simulink model "rc_receiver"  (R2026b)
settings: Solver=VariableStepAuto
undefined symbols (not defined in the file or in its folder): DiscIntNeverNeededParam, P, Ts
libraries: simulink x1
settings Model: Creator=aomar  LastModifiedBy=aomar

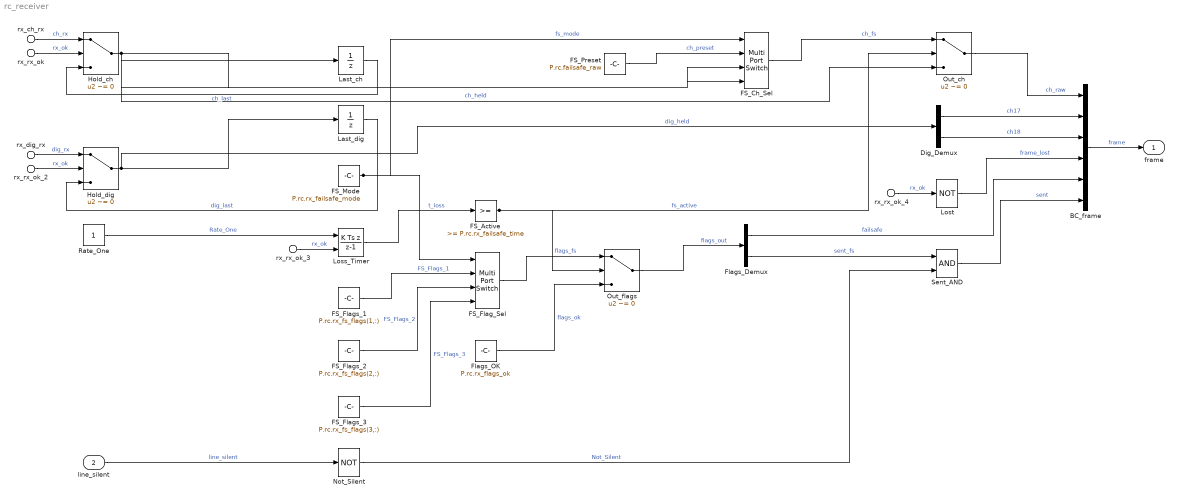
== system rc_receiver ==
  rx_ch_rx : Inport  PortName=rx  Element=ch_rx
  rx_rx_ok : Inport  PortName=rx  Element=rx_ok
  rx_rx_ok_2 : Inport  PortName=rx  Element=rx_ok
  rx_rx_ok_3 : Inport  PortName=rx  Element=rx_ok
  rx_rx_ok_4 : Inport  PortName=rx  Element=rx_ok
  rx_dig_rx : Inport  PortName=rx  Element=dig_rx
  line_silent : Inport  Port=2  OutDataTypeStr=boolean  PortDimensions=1  SampleTime=Ts.rc_frame
  BC_frame : BusCreator  Inputs=6  OutDataTypeStr=Bus: Bus_RcFrame  NonVirtualBus=on
      settings: InheritFromInputs=off
  Dig_Demux : Demux  Outputs=2
  FS_Active : simulink/Logic and Bit Operations/Compare To Constant  relop=>=  const=P.rc.rx_failsafe_time  OutDataTypeStr=boolean
  FS_Ch_Sel : MultiPortSwitch  SaturateOnIntegerOverflow=off  InputSameDT=off
  FS_Flag_Sel : MultiPortSwitch  SaturateOnIntegerOverflow=off  InputSameDT=off
  FS_Flags_1 : Constant  Value=P.rc.rx_fs_flags(1,:)  OutDataTypeStr=boolean  SampleTime=Ts.rc_frame
  FS_Flags_2 : Constant  Value=P.rc.rx_fs_flags(2,:)  OutDataTypeStr=boolean  SampleTime=Ts.rc_frame
  FS_Flags_3 : Constant  Value=P.rc.rx_fs_flags(3,:)  OutDataTypeStr=boolean  SampleTime=Ts.rc_frame
  FS_Mode : Constant  Value=P.rc.rx_failsafe_mode  SampleTime=Ts.rc_frame
  FS_Preset : Constant  Value=P.rc.failsafe_raw  OutDataTypeStr=uint16  SampleTime=Ts.rc_frame
  Flags_Demux : Demux  Outputs=2
  Flags_OK : Constant  Value=P.rc.rx_flags_ok  OutDataTypeStr=boolean  SampleTime=Ts.rc_frame
  Hold_ch : Switch  Criteria=u2 ~= 0  SaturateOnIntegerOverflow=off  InputSameDT=off
  Hold_dig : Switch  Criteria=u2 ~= 0  SaturateOnIntegerOverflow=off  InputSameDT=off
  Last_ch : UnitDelay  InitialCondition=P.rc.failsafe_raw  SampleTime=Ts.rc_frame
  Last_dig : UnitDelay  SampleTime=Ts.rc_frame
  Loss_Timer : DiscreteIntegrator  IntegratorMethod=Integration: Backward Euler  gainval=1  ExternalReset=level  SampleTime=Ts.rc_frame  LimitOutput=on  UpperSaturationLimit=P.rc.rx_timer_sat  LowerSaturationLimit=0  ICPrevOutput=DiscIntNeverNeededParam  ICPrevScaledInput=DiscIntNeverNeededParam
  Lost : Logic  Operator=NOT  Inputs=1  AllPortsSameDT=off  OutDataTypeStr=boolean
  Not_Silent : Logic  Operator=NOT  Inputs=1  AllPortsSameDT=off  OutDataTypeStr=boolean
  Out_ch : Switch  Criteria=u2 ~= 0  SaturateOnIntegerOverflow=off  InputSameDT=off
  Out_flags : Switch  Criteria=u2 ~= 0  SaturateOnIntegerOverflow=off  InputSameDT=off
  Rate_One : Constant  SampleTime=Ts.rc_frame
  Sent_AND : Logic  AllPortsSameDT=off  OutDataTypeStr=boolean
  frame : Outport  OutDataTypeStr=Bus: Bus_RcFrame  SampleTime=Ts.rc_frame
  wires:
  rx_ch_rx/1 -> Hold_ch/1  "ch_rx"
  rx_rx_ok/1 -> Hold_ch/2  "rx_ok"
  rx_dig_rx/1 -> Hold_dig/1  "dig_rx"
  rx_rx_ok_2/1 -> Hold_dig/2  "rx_ok"
  Rate_One/1 -> Loss_Timer/1  "Rate_One"
  line_silent/1 -> Not_Silent/1  "line_silent"
  Hold_ch/1 -> FS_Ch_Sel/4, FS_Ch_Sel/3, Out_ch/3, Last_ch/1  "ch_held"
  Hold_dig/1 -> Last_dig/1, Dig_Demux/1  "dig_held"
  rx_rx_ok_3/1 -> Loss_Timer/2  "rx_ok"
  FS_Mode/1 -> FS_Ch_Sel/1, FS_Flag_Sel/1  "fs_mode"
  FS_Flags_1/1 -> FS_Flag_Sel/2  "FS_Flags_1"
  FS_Flags_2/1 -> FS_Flag_Sel/3  "FS_Flags_2"
  FS_Flags_3/1 -> FS_Flag_Sel/4  "FS_Flags_3"
  Not_Silent/1 -> Sent_AND/2  "Not_Silent"
  Last_ch/1 -> Hold_ch/3  "ch_last"
  Last_dig/1 -> Hold_dig/3  "dig_last"
  Loss_Timer/1 -> FS_Active/1  "t_loss"
  FS_Active/1 -> Out_ch/2, Out_flags/2  "fs_active"
  Flags_OK/1 -> Out_flags/3  "flags_ok"
  FS_Flag_Sel/1 -> Out_flags/1  "flags_fs"
  FS_Preset/1 -> FS_Ch_Sel/2  "ch_preset"
  Out_flags/1 -> Flags_Demux/1  "flags_out"
  Flags_Demux/1 -> BC_frame/5  "failsafe"
  Flags_Demux/2 -> Sent_AND/1  "sent_fs"
  FS_Ch_Sel/1 -> Out_ch/1  "ch_fs"
  rx_rx_ok_4/1 -> Lost/1  "rx_ok"
  Dig_Demux/1 -> BC_frame/2  "ch17"
  Dig_Demux/2 -> BC_frame/3  "ch18"
  Lost/1 -> BC_frame/4  "frame_lost"
  Sent_AND/1 -> BC_frame/6  "sent"
  Out_ch/1 -> BC_frame/1  "ch_raw"
  BC_frame/1 -> frame/1  "frame"
